simulink model "gantry_home_center"  (R2025b)
settings: Solver=FixedStepDiscrete  StartTime=0.0  StopTime=inf  FixedStep=0.05  RelTol=1e-3  EnableMultiTasking=on
libraries: raspberrypiBasiclib x4, simulink x2, raspberrypiNetworklib x1
settings Model: Creator=jeets  LastModifiedBy=jeets
settings SolverCC: PositivePriorityOrder=on
settings OptimizationCC: EnhancedBackFolding=on  PassReuseOutputArgsAs=Individual arguments  ZeroExternalMemoryAtStartup=off  ZeroInternalMemoryAtStartup=off  MaxStackSize=200000  OptimizeBlockOrder=speed  DifferentSizesBufferReuse=on  OptimizationCustomize=off  EfficientTunableParamExpr=on
settings DebuggingCC: ParameterTunabilityLossMsg=error
settings HardwareCC: ProdBitPerPointer=32.0  ProdBitPerSizeT=32.0  ProdBitPerPtrDiffT=32.0  ProdLargestAtomicInteger=Long  ProdLargestAtomicFloat=Double  ProdWordSize=32.0  ProdLongLongMode=on  ProdHWDeviceType=ARM Compatible->ARM Cortex-A (32-bit)
settings RTWCC: SystemTargetFile=ert.tlc  HardwareBoard=Raspberry Pi  TLCOptions="-aInlineSetEventsForThisBaseRateFcn=TLC_FALSE -aSuppressMultiTaskScheduler=TLC_FALSE  -aRateBasedStepFcn=0"  TemplateMakefile=ert_default_tmf  Toolchain=GNU GCC Embedded Linux  BuildConfiguration=Faster Runs  Description=Embedded Coder
settings CodeAppCC: ForceParamTrailComments=on  IgnoreCustomStorageClasses=off  OperatorAnnotations=on  SimulinkDataObjDesc=on  SFDataObjDesc=on  InsertBlockDesc=on
settings ERTTargetCC: ExtModeTransport=2.0  ExtModeStaticAlloc=on  ExtModeMexFile=ext_xcp  ExtModeIntrfLevel=Level2 - Open  InlinedParameterPlacement=Hierarchical  CodeReplacementLibrary=ARM Cortex-A CMSIS  SupportVariableSizeSignals=on

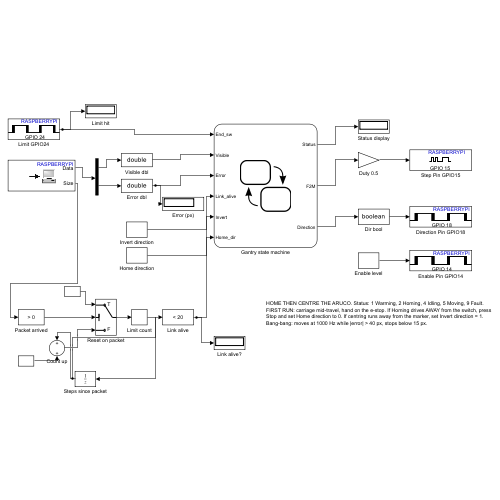
[thumbnail: Simulink's stored preview of the top-level diagram]
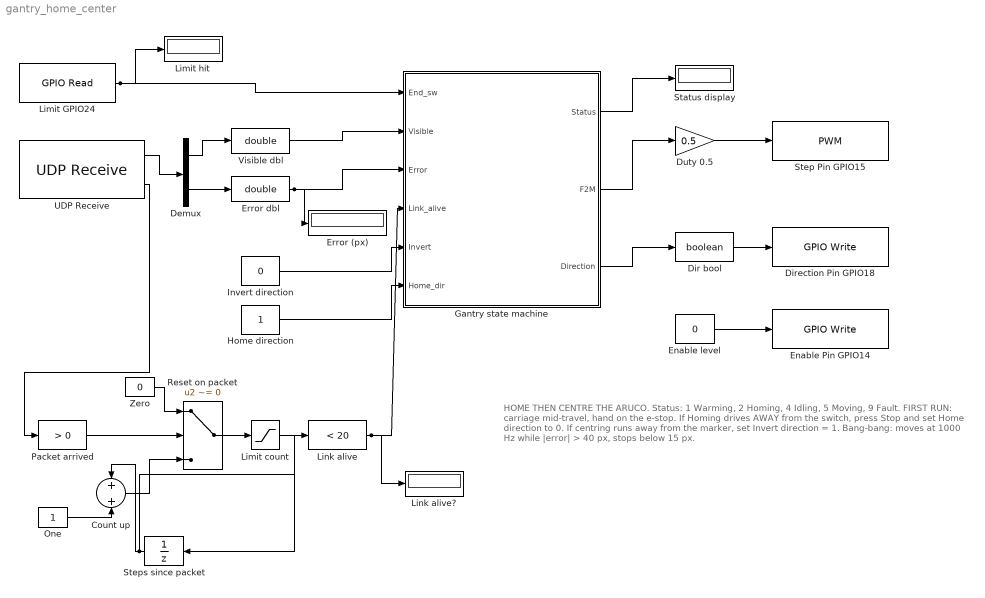
== system gantry_home_center ==
  note: HOME THEN CENTRE THE ARUCO. Status: 1 Warming, 2 Homing, 4 Idling, 5 Moving, 9 Fault.
      | FIRST RUN: carriage mid-travel, hand on the e-stop. If Homing drives AWAY from the switch, press
      | Stop and set Home direction to 0. If centring runs away from the marker, set Invert direction = 1.
      | Bang-bang: moves at 1000 Hz while |error| > 40 px, stops below 15 px.
  Count up : Sum
  Demux : Demux  Outputs=2
  Dir bool : DataTypeConversion  OutDataTypeStr=boolean  SaturateOnIntegerOverflow=off  RndMeth=Floor
  Direction Pin GPIO18 : raspberrypiBasiclib/GPIO Write  BoardProperty=Pi 3 Model B+  gpio=18  blockPlatform=Raspberry Pi  PinNumber=17  board=[]  direction=[]
  Duty 0.5 : Gain  Gain=0.5
  Enable Pin GPIO14 : raspberrypiBasiclib/GPIO Write  BoardProperty=Pi 3 Model B+  gpio=14  blockPlatform=Raspberry Pi  PinNumber=17  board=[]  direction=[]
  Enable level : Constant  Value=0  OutDataTypeStr=boolean
  Error (px) : Display
  Error dbl : DataTypeConversion  OutDataTypeStr=double  SaturateOnIntegerOverflow=off  RndMeth=Floor
  Gantry state machine : Stateflow chart  TreatAsAtomicUnit=on
  Home direction : Constant
  Invert direction : Constant  Value=0
  Limit GPIO24 : raspberrypiBasiclib/GPIO Read  BoardProperty=Pi 3 Model B+  gpio=24  SampleTime=0.05  blockPlatform=Raspberry Pi  PinNumber=4  board=[]  direction=[]  internalResistor=[]
  Limit count : Saturate  UpperLimit=1000  LowerLimit=0
  Limit hit : Display
  Link alive : simulink/Logic and Bit Operations/Compare To Constant  relop=<  const=20  OutDataTypeStr=boolean
  Link alive? : Display
  One : Constant
  Packet arrived : simulink/Logic and Bit Operations/Compare To Zero  relop=>  OutDataTypeStr=boolean
  Reset on packet : Switch  Criteria=u2 ~= 0  SaturateOnIntegerOverflow=off  InputSameDT=off
  Status display : Display
  Step Pin GPIO15 : raspberrypiBasiclib/PWM  board=Pi 3 Model B+  Pin_=15  Frequency=1000  blockPlatform=Raspberry Pi
  Steps since packet : UnitDelay  InitialCondition=20  SampleTime=0.05  HasFrameUpgradeWarning=on
  UDP Receive : raspberrypiNetworklib/UDP Receive  localURL='0.0.0.0'  localPort=50001  remoteURL='0.0.0.0'  remotePort=-1  recvBufferSize=8192  signalDatatype=int16  dims=2  isVarSize=off  showBlockingTime=off  blockingTime=0  sampletime=0.05  blockPlatform=Raspberry Pi
  Visible dbl : DataTypeConversion  OutDataTypeStr=double  SaturateOnIntegerOverflow=off  RndMeth=Floor
  Zero : Constant  Value=0
  wires:
  Limit GPIO24/1 -> Gantry state machine/1(End_sw), Limit hit/1
  UDP Receive/1 -> Demux/1
  Demux/1 -> Visible dbl/1
  Visible dbl/1 -> Gantry state machine/2(Visible)
  Demux/2 -> Error dbl/1
  Error dbl/1 -> Gantry state machine/3(Error), Error (px)/1
  Link alive/1 -> Gantry state machine/4(Link_alive), Link alive?/1
  Invert direction/1 -> Gantry state machine/5(Invert)
  Home direction/1 -> Gantry state machine/6(Home_dir)
  Gantry state machine/1(Status) -> Status display/1
  Gantry state machine/2(F2M) -> Duty 0.5/1
  Duty 0.5/1 -> Step Pin GPIO15/1
  Gantry state machine/3(Direction) -> Dir bool/1
  Dir bool/1 -> Direction Pin GPIO18/1
  Enable level/1 -> Enable Pin GPIO14/1
  UDP Receive/2 -> Packet arrived/1
  Zero/1 -> Reset on packet/1
  Packet arrived/1 -> Reset on packet/2
  Count up/1 -> Reset on packet/3
  Reset on packet/1 -> Limit count/1
  Limit count/1 -> Steps since packet/1
  Steps since packet/1 -> Count up/1, Link alive/1
  One/1 -> Count up/2

== stateflow chart gantry_home_center/Gantry state machine ==
  settings: updateMethod=DISCRETE  sampleTime=0.05
  state Warming
    en:
    Status = 1;
    F2M = 0;
  state Homing
    en:
    Status = 2;
    Direction = Home_dir;
    F2M = 1;
  state Fault
    en:
    Status = 9;
    F2M = 0;
  state Idling
    en:
    Status = 4;
    F2M = 0;
  state Moving
    en, du:
    Status = 5;
    Direction = double(xor(Error > 0, Invert ~= 0));
    F2M = 1;
  (default) -> Warming
  Warming -> Homing : after(5,sec)
  Homing -> Fault [order 2] : after(60,sec)
  Moving -> Idling : [~Link_alive || ~Visible || abs(Error) < 15 || (End_sw == 1 && Direction == Home_dir)]
  Homing -> Idling [order 1] : [End_sw == 1]
  Idling -> Moving : [Link_alive && Visible && abs(Error) > 40 && ~(End_sw == 1 && double(xor(Error > 0, Invert ~= 0)) == Home_dir)]
  data: End_sw input; Visible input; Error input; Link_alive input; Invert input; Home_dir input; Status output double; F2M output double; Direction output double
